simulink library "Lib_Piccolo"  (R2018b)
settings: Solver=VariableStepAuto  StartTime=0.0  StopTime=10.0  RelTol=1e-3
values from neighbouring files (symbols this model uses):
  AccelErrInt2Brakes = 0.15    [SimulationControlConfig16P.m]    (also in SimulationControlConfig16P_LEGACY.m; SimulationControlConfigTAILLESS.m = 0.2; SimulationControlConfigUTAIL.m = 0.2)
  AileronMax = 25    [SimulationControlConfig16P.m]    (also in SimulationControlConfig16P_LEGACY.m; SimulationControlConfigTAILLESS.m; SimulationControlConfigUTAIL.m)
  AileronPower = 0.00268    [SimulationControlConfig16P.m]    (also in SimulationControlConfig16P_LEGACY.m; SimulationControlConfigTAILLESS.m; SimulationControlConfigUTAIL.m)
  AileronSurfaceMax = 45    [SimulationControlConfig16P.m]    (also in SimulationControlConfig16P_LEGACY.m)
  AileronTrim = 0    [SimulationControlConfig16P.m]    (also in SimulationControlConfig16P_LEGACY.m; SimulationControlConfigTAILLESS.m; SimulationControlConfigUTAIL.m)
  Alt = 1000 + TerrainHeight    [SimulationStateConfig.m]
  AltCruise_m = testPlans(testIndx).terrainElevation * 0.3048 + 200    [SimulationControlConfig16P.m]    (also in SimulationControlConfigTAILLESS.m = 1083; SimulationControlConfigUTAIL.m = testPlans(testIndx).terrainElevation * 0.3048 + 152)
  AltitudeRate2PitchCmdIntegratorInit = 0.1    [SimulationControlPre.m]
  AltMax = 10000    [SimulationControlConfig16P.m]    (also in SimulationControlConfig16P_LEGACY.m; SimulationControlConfigTAILLESS.m; SimulationControlConfigUTAIL.m)
  AltMaxAccel = 1.25    [SimulationControlConfig16P.m]    (also in SimulationControlConfig16P_LEGACY.m = 0.9; SimulationControlConfigTAILLESS.m = 1.7; SimulationControlConfigUTAIL.m = 2)
  AltMin = 0    [SimulationControlConfig16P.m]    (also in SimulationControlConfig16P_LEGACY.m; SimulationControlConfigTAILLESS.m; SimulationControlConfigUTAIL.m)
  AltRateCmd2Pitch = 0.50    (= 0.5)    [SimulationControlConfig16P.m]    (also in SimulationControlConfig16P_LEGACY.m = 0.6; SimulationControlConfigTAILLESS.m = 0.2; SimulationControlConfigUTAIL.m = 0.3)
  AltRateError2Pitch = 0.40    (= 0.4)    [SimulationControlConfig16P.m]    (also in SimulationControlConfig16P_LEGACY.m; SimulationControlConfigTAILLESS.m = 0.55; SimulationControlConfigUTAIL.m = 0.55)
  AltRateErrorInt2Pitch = 0.50    (= 0.5)    [SimulationControlConfig16P.m]    (also in SimulationControlConfig16P_LEGACY.m = 0.45; SimulationControlConfigTAILLESS.m; SimulationControlConfigUTAIL.m = 0.75)
  AltRateLpfCutOff = 3    [SimulationControlConfig16P.m]    (also in SimulationControlConfig16P_LEGACY.m; SimulationControlConfigTAILLESS.m = 2; SimulationControlConfigUTAIL.m = 2)
  AutoNosegear2Rudder = 26    [SimulationControlConfig16P.m]    (also in SimulationControlConfig16P_LEGACY.m; SimulationControlConfigTAILLESS.m = 25.2; SimulationControlConfigUTAIL.m = 14)
  b = 5.54    [SimulationControlConfig16P.m]    (also in SimulationControlConfig16P_LEGACY.m; SimulationControlConfigTAILLESS.m = 2.37; SimulationControlConfigUTAIL.m = 2.37)
  Bank2AileronIntegratorInit = 0    [SimulationControlPre.m]
  BankMax_User = BankMax_User/180*pi    (= 0.523598775598)    [SimulationControlConfig16P.m]    (also in SimulationControlConfig16P_LEGACY.m; SimulationControlConfigTAILLESS.m = 0.610865238198; SimulationControlConfigUTAIL.m = 0.628318530718)
  baseLegFlaps = 20    [SimulationControlConfig16P.m]    (also in SimulationControlConfig16P_LEGACY.m = 0; SimulationControlConfigTAILLESS.m = 15; SimulationControlConfigUTAIL.m = 10)
  C = GeneticOpt.C    [SimulationCostFunction.m]
  c = Sw/b    (= 0.841696750903)    [SimulationControlConfig16P.m]    (also in SimulationControlConfig16P_LEGACY.m; SimulationControlConfigTAILLESS.m = 0.354008438819; SimulationControlConfigUTAIL.m = 0.354008438819)
  cell2WheelFactorMG = 5.98    [SimulationSensorConfig16P_LEGACY.m]
  cell2WheelFactorNG = 1    [SimulationSensorConfig16P_LEGACY.m]
  cellSatMaxMG = 15000    [SimulationSensorConfig16P.m]    (also in SimulationSensorConfig16P_LEGACY.m; SimulationSensorConfigTAILLESS7P.m; SimulationSensorConfigUTAIL7P.m)
  cellSatMaxNG = 1000    [SimulationSensorConfig16P.m]    (also in SimulationSensorConfig16P_LEGACY.m; SimulationSensorConfigTAILLESS7P.m; SimulationSensorConfigUTAIL7P.m)
  cellSatMinMG = -15000    [SimulationSensorConfig16P.m]    (also in SimulationSensorConfig16P_LEGACY.m; SimulationSensorConfigTAILLESS7P.m; SimulationSensorConfigUTAIL7P.m)
  cellSatMinNG = -1000    [SimulationSensorConfig16P.m]    (also in SimulationSensorConfig16P_LEGACY.m; SimulationSensorConfigTAILLESS7P.m; SimulationSensorConfigUTAIL7P.m)
  CL_Limit = CL_Max    (= 0.54)    [SimulationControlConfig16P.m]    (also in SimulationControlConfig16P_LEGACY.m; SimulationControlConfigTAILLESS.m; SimulationControlConfigUTAIL.m = 0.53)
  CL_Max = 0.54    [SimulationControlConfig16P.m]    (also in SimulationControlConfig16P_LEGACY.m; SimulationControlConfigTAILLESS.m; SimulationControlConfigUTAIL.m = 0.53)
  CL_Max_Nom = 0.465    [SimulationControlConfig16P.m]    (also in SimulationControlConfig16P_LEGACY.m; SimulationControlConfigTAILLESS.m = 0.39; SimulationControlConfigUTAIL.m)
  CL_Min = 0    [SimulationControlConfig16P.m]    (also in SimulationControlConfig16P_LEGACY.m; SimulationControlConfigTAILLESS.m; SimulationControlConfigUTAIL.m)
  ClimbMaxFraction = 0.35    [SimulationControlConfig16P.m]    (also in SimulationControlConfig16P_LEGACY.m = 0.24; SimulationControlConfigTAILLESS.m = 0.19; SimulationControlConfigUTAIL.m = 0.21)
  ClimboutMaxBank = 7.0    (= 7)    [SimulationControlConfig16P.m]    (also in SimulationControlConfig16P_LEGACY.m; SimulationControlConfigTAILLESS.m = 5; SimulationControlConfigUTAIL.m)
  ClimboutTimer = 7.0    (= 7)    [SimulationControlConfig16P.m]    (also in SimulationControlConfig16P_LEGACY.m; SimulationControlConfigTAILLESS.m; SimulationControlConfigUTAIL.m)
  dCl_per_dFlap = 0.005581818    [SimulationControlConfig16P.m]    (also in SimulationControlConfig16P_LEGACY.m = 0; SimulationControlConfigTAILLESS.m = 0; SimulationControlConfigUTAIL.m = 0)
  DecelerationCmd = 3.1    [SimulationControlConfig16P.m]    (also in SimulationControlConfig16P_LEGACY.m; SimulationControlConfigTAILLESS.m = 0.1; SimulationControlConfigUTAIL.m = 0.1)
  DeRotateLogicEndTimer = abs((NoseDownLimit_Deg-1)/DeRotateRamp_Dps)    [SimulationControlConfig16P.m]    (also in SimulationControlConfig16P_LEGACY.m; SimulationControlConfigTAILLESS.m; SimulationControlConfigUTAIL.m)
  DeRotateLogicHoldNoseUpTimer = 0.1    [SimulationControlConfig16P.m]    (also in SimulationControlConfig16P_LEGACY.m; SimulationControlConfigTAILLESS.m; SimulationControlConfigUTAIL.m)
  DeRotateLogicTimerTimeout = 2    [SimulationControlConfig16P.m]    (also in SimulationControlConfig16P_LEGACY.m; SimulationControlConfigTAILLESS.m; SimulationControlConfigUTAIL.m)
  DeRotateLowerCmdSaturation = 0    [SimulationControlConfig16P.m]    (also in SimulationControlConfig16P_LEGACY.m; SimulationControlConfigTAILLESS.m; SimulationControlConfigUTAIL.m)
  DeRotateRamp_Dps = 3    [SimulationControlConfig16P.m]    (also in SimulationControlConfig16P_LEGACY.m; SimulationControlConfigTAILLESS.m = 8; SimulationControlConfigUTAIL.m = 8)
  DeRotateUpperCmdSaturation = 7    [SimulationControlConfig16P.m]    (also in SimulationControlConfig16P_LEGACY.m; SimulationControlConfigTAILLESS.m; SimulationControlConfigUTAIL.m)
  DescentMaxFraction = 0.22    [SimulationControlConfig16P.m]    (also in SimulationControlConfig16P_LEGACY.m = 0.2; SimulationControlConfigTAILLESS.m = 0.17; SimulationControlConfigUTAIL.m = 0.17)
  DesktopSimTerrainOffset_m = 0.406    [SimulationAircraftConfig.m]
  downwindFlaps = 0    [SimulationControlConfig16P.m]    (also in SimulationControlConfig16P_LEGACY.m; SimulationControlConfigTAILLESS.m; SimulationControlConfigUTAIL.m)
  DP_init = 0.5*1.225*V_init^2    [SimulationControlConfig16P.m]    (also in SimulationControlConfig16P_LEGACY.m; SimulationControlConfigTAILLESS.m; SimulationControlConfigUTAIL.m)
  dscNoiseMG = 1    [SimulationSensorConfig16P_LEGACY.m]
  dscNoiseNG = 0.25    [SimulationSensorConfig16P_LEGACY.m]
  DSCnumBits = 24    [SimulationSensorConfig16P.m]    (also in SimulationSensorConfig16P_LEGACY.m; SimulationSensorConfigTAILLESS7P.m; SimulationSensorConfigUTAIL7P.m)
  DSCRangeMaxMG = 15000    [SimulationSensorConfig16P.m]    (also in SimulationSensorConfig16P_LEGACY.m; SimulationSensorConfigTAILLESS7P.m; SimulationSensorConfigUTAIL7P.m)
  DSCRangeMaxNG = 1000    [SimulationSensorConfig16P.m]    (also in SimulationSensorConfig16P_LEGACY.m; SimulationSensorConfigTAILLESS7P.m; SimulationSensorConfigUTAIL7P.m)
  DSCRangeMinMG = -15000    [SimulationSensorConfig16P.m]    (also in SimulationSensorConfig16P_LEGACY.m; SimulationSensorConfigTAILLESS7P.m; SimulationSensorConfigUTAIL7P.m)
  DSCRangeMinNG = -1000    [SimulationSensorConfig16P.m]    (also in SimulationSensorConfig16P_LEGACY.m; SimulationSensorConfigTAILLESS7P.m; SimulationSensorConfigUTAIL7P.m)
  dt = DLLSim.dt    [SimulationTimeStep.m]    (also in SimulationTrim.m = 0.02)
  EarlyTouchdownThreshold = 3.0    (= 3)    [SimulationControlConfig16P.m]    (also in SimulationControlConfig16P_LEGACY.m; SimulationControlConfigTAILLESS.m = 2.2; SimulationControlConfigUTAIL.m = 2.5)
  ElevatorDeflectionRate = 15    [SimulationControlConfig16P.m]    (also in SimulationControlConfig16P_LEGACY.m = 12; SimulationControlConfigTAILLESS.m = 10; SimulationControlConfigUTAIL.m = 12)
  ElevatorMax = 25    [SimulationControlConfig16P.m]    (also in SimulationControlConfig16P_LEGACY.m; SimulationControlConfigTAILLESS.m; SimulationControlConfigUTAIL.m)
  ElevatorPower = -0.002209    [SimulationControlConfig16P.m]    (also in SimulationControlConfig16P_LEGACY.m; SimulationControlConfigTAILLESS.m = -0.002956; SimulationControlConfigUTAIL.m = -0.00205983)
  ElevatorTrim = -3.5    [SimulationControlConfig16P.m]    (also in SimulationControlConfig16P_LEGACY.m; SimulationControlConfigTAILLESS.m = -6; SimulationControlConfigUTAIL.m = -8)
  elevonBias = 0    [SimulationControlConfig16P.m]    (also in SimulationControlConfig16P_LEGACY.m; SimulationControlConfigTAILLESS.m; SimulationControlConfigUTAIL.m)
  Enable_TAS_Protection = 0    [SimulationControlConfig16P.m]    (also in SimulationControlConfig16P_LEGACY.m; SimulationControlConfigTAILLESS.m; SimulationControlConfigUTAIL.m)
  EnableCrossTrackAbort = 1    [SimulationControlConfig16P.m]    (also in SimulationControlConfigTAILLESS.m; SimulationControlConfigUTAIL.m)
  EnergyBandwidth = 0.02    [SimulationControlConfig16P.m]    (also in SimulationControlConfig16P_LEGACY.m; SimulationControlConfigTAILLESS.m = 0.06; SimulationControlConfigUTAIL.m = 0.06)
  EngineLhFuelCut = 0    [SimulationAircraftConfig.m]
  EngineRhFuelCut = 0    [SimulationAircraftConfig.m]
  FastThrottleRate = 0.075    [SimulationControlConfig16P.m]    (also in SimulationControlConfig16P_LEGACY.m = 0.05; SimulationControlConfigTAILLESS.m = 0.1; SimulationControlConfigUTAIL.m = 0.1)
  FilterWarmUpTime = 2    [SimulationSensorConfig16P.m]    (also in SimulationSensorConfig16P_LEGACY.m; SimulationSensorConfigTAILLESS7P.m; SimulationSensorConfigUTAIL7P.m)
  finalApproachFlaps = 20    [SimulationControlConfig16P.m]    (also in SimulationControlConfig16P_LEGACY.m = 0; SimulationControlConfigTAILLESS.m = 22; SimulationControlConfigUTAIL.m = 10)
  FinalDescentSlope_Deg = testPlans(testIndx).descentSlope    [SimulationControlConfig16P.m]    (also in SimulationControlConfig16P_LEGACY.m; SimulationControlConfigTAILLESS.m; SimulationControlConfigUTAIL.m)
  flapMax = 0    [SimulationControlConfig16P.m]    (also in SimulationControlConfig16P_LEGACY.m; SimulationControlConfigTAILLESS.m; SimulationControlConfigUTAIL.m)
  flapRate = 7.5    [SimulationControlConfig16P.m]    (also in SimulationControlConfig16P_LEGACY.m; SimulationControlConfigTAILLESS.m = 6.6; SimulationControlConfigUTAIL.m)
  FlareHeight = 5    [SimulationControlConfig16P.m]    (also in SimulationControlConfig16P_LEGACY.m = 4.8; SimulationControlConfigTAILLESS.m = 2.5; SimulationControlConfigUTAIL.m = 2)
  FlareVerticalRate_mps = -0.4    [SimulationControlConfig16P.m]    (also in SimulationControlConfig16P_LEGACY.m = -0.5; SimulationControlConfigTAILLESS.m = -0.15; SimulationControlConfigUTAIL.m = -0.15)
  Fp_Aileron = 0.55*2*pi*RollRateLpfCutoff*dt    [SimulationControlConfig16P.m]    (also in SimulationControlConfig16P_LEGACY.m; SimulationControlConfigTAILLESS.m; SimulationControlConfigUTAIL.m)
  Fp_Alt = 0.55*AltBandwidth    (= 0.099)    [SimulationControlConfig16P.m]    (also in SimulationControlConfig16P_LEGACY.m; SimulationControlConfigTAILLESS.m = 0.587477826221; SimulationControlConfigUTAIL.m = 0.69115038379)
  Fp_AltRate = 0.55*2*pi*AltRateLpfCutOff*dt    [SimulationControlConfig16P.m]    (also in SimulationControlConfig16P_LEGACY.m; SimulationControlConfigTAILLESS.m; SimulationControlConfigUTAIL.m)
  Fp_Elevator = 0.55*2*pi*PitchRateLpfCutoff*dt    [SimulationControlConfig16P.m]    (also in SimulationControlConfig16P_LEGACY.m; SimulationControlConfigTAILLESS.m; SimulationControlConfigUTAIL.m)
  Fp_Energy = 0.55*2*pi*EnergyBandwidth    (= 0.069115038379)    [SimulationControlConfig16P.m]    (also in SimulationControlConfig16P_LEGACY.m; SimulationControlConfigTAILLESS.m = 0.207345115137; SimulationControlConfigUTAIL.m = 0.207345115137)
  Fp_Energy2 = 0.55*2*pi*EnergyBandwidth*dt    [SimulationControlConfig16P.m]    (also in SimulationControlConfig16P_LEGACY.m; SimulationControlConfigTAILLESS.m; SimulationControlConfigUTAIL.m)
  Fp_Pitch = 0.55*2*pi*PitchBandwidth    (= 2.76460153516)    [SimulationControlConfig16P.m]    (also in SimulationControlConfig16P_LEGACY.m = 3.11017672705; SimulationControlConfigTAILLESS.m = 3.80132711084; SimulationControlConfigUTAIL.m = 2.41902634326)
  Fp_Pitch_2 = 0.55*2*pi*PitchBandwidth*dt    [SimulationControlConfig16P.m]    (also in SimulationControlConfig16P_LEGACY.m; SimulationControlConfigTAILLESS.m; SimulationControlConfigUTAIL.m)
  Fp_Roll = RollBandwidth^2    (= 1)    [SimulationControlConfig16P.m]    (also in SimulationControlConfig16P_LEGACY.m = 1.44; SimulationControlConfigTAILLESS.m; SimulationControlConfigUTAIL.m)
  Fp_Rudder = 0.55*2*pi*YawRateLpfCutoff*dt    [SimulationControlConfig16P.m]    (also in SimulationControlConfig16P_LEGACY.m; SimulationControlConfigTAILLESS.m; SimulationControlConfigUTAIL.m)
  Fp_TAS = 0.55*2*pi*TASBandwidth    (= 0.103672557568)    [SimulationControlConfig16P.m]    (also in SimulationControlConfig16P_LEGACY.m; SimulationControlConfigTAILLESS.m = 0.172787595947; SimulationControlConfigUTAIL.m = 0.172787595947)
  Fp_TAS_Filter = 2*pi*TasLpfCutoff*dt    [SimulationControlConfig16P.m]    (also in SimulationControlConfig16P_LEGACY.m; SimulationControlConfigTAILLESS.m; SimulationControlConfigUTAIL.m)
  Fp_Turn = 0.55*2*pi*TurnErrLPFcutoff    (= 0.0345575191895)    [SimulationControlConfig16P.m]    (also in SimulationControlConfig16P_LEGACY.m; SimulationControlConfigTAILLESS.m = 0.172787595947; SimulationControlConfigUTAIL.m = 0.172787595947)
  Fp_TurnDerr = 0.55*2*pi*TurnDerivativeLPFcutoff    (= 0.0345575191895)    [SimulationControlConfig16P.m]    (also in SimulationControlConfig16P_LEGACY.m; SimulationControlConfigTAILLESS.m = 0.172787595947; SimulationControlConfigUTAIL.m = 0.172787595947)
  FTV = 3    [SimulationAircraftConfig.m]
  ftvStaticPositionError = 1/1.18    (= 0.847457627119)    [SimulationSensorConfig16P.m]    (also in SimulationSensorConfig16P_LEGACY.m; SimulationSensorConfigTAILLESS7P.m = 1; SimulationSensorConfigUTAIL7P.m = 1)
  g = 9.81    [SimulationStateConfig.m]
  GustSpd_Kts = testPlans(testIndx).gustSpd    [SimulationStateConfig.m]
  GustTriggerVal = testPlans(testIndx).gustTriggerVal    [SimulationStateConfig.m]
  HeadingErr2TurnRate = 0.5    [SimulationControlConfig16P.m]    (also in SimulationControlConfig16P_LEGACY.m; SimulationControlConfigTAILLESS.m; SimulationControlConfigUTAIL.m)
  HeadingErrDer2TurnRate = 0.3    [SimulationControlConfig16P.m]    (also in SimulationControlConfig16P_LEGACY.m; SimulationControlConfigTAILLESS.m; SimulationControlConfigUTAIL.m)
  IASbounce = IASstall*0.8    [SimulationControlPre.m]
  IAScruiseCMD = sqrt(2*m*9.81/(1.225*Sw*CL_cruise))    [SimulationControlConfig16P.m]    (also in SimulationControlConfig16P_LEGACY.m; SimulationControlConfigTAILLESS.m; SimulationControlConfigUTAIL.m)
  IASfinalCMD = 1.12 * IASmin    [SimulationControlConfig16P.m]    (also in SimulationControlConfig16P_LEGACY.m = 1.10 * IASmin; SimulationControlConfigTAILLESS.m = 1.10 * IASmin; SimulationControlConfigUTAIL.m = 1.15 * IASmin)
  IASflareCMD = IASstall    [SimulationControlConfig16P.m]    (also in SimulationControlConfig16P_LEGACY.m; SimulationControlConfigTAILLESS.m; SimulationControlConfigUTAIL.m)
  IASmax = 64    [SimulationControlConfig16P.m]    (also in SimulationControlConfig16P_LEGACY.m = 46; SimulationControlConfigTAILLESS.m = 38.58; SimulationControlConfigUTAIL.m = 35)
  IASmin = sqrt(2*m*9.81/(1.225*Sw*0.9*CL_Max_Nom))    [SimulationControlConfig16P.m]    (also in SimulationControlConfig16P_LEGACY.m; SimulationControlConfigTAILLESS.m; SimulationControlConfigUTAIL.m)
  IASshortCMD = IASstall    [SimulationControlConfig16P.m]    (also in SimulationControlConfig16P_LEGACY.m; SimulationControlConfigTAILLESS.m; SimulationControlConfigUTAIL.m)
  IASstall = sqrt(2*m*9.81/(1.225*Sw*CL_Max))    [SimulationControlConfig16P.m]    (also in SimulationControlConfig16P_LEGACY.m; SimulationControlConfigTAILLESS.m; SimulationControlConfigUTAIL.m)
  inFlight = 1    [SimulationControlConfig16P.m]    (also in SimulationControlConfigTAILLESS.m; SimulationControlConfigUTAIL.m)
  JetCatOffset = 5    [SimulationControlConfig16P.m]    (also in SimulationControlConfig16P_LEGACY.m)
  LaunchRollingElevator = -1.5    [SimulationControlConfig16P.m]    (also in SimulationControlConfig16P_LEGACY.m; SimulationControlConfigTAILLESS.m = 1; SimulationControlConfigUTAIL.m = 1)
  ldg_NosegearMax = 10    [SimulationControlConfig16P.m]    (also in SimulationControlConfig16P_LEGACY.m; SimulationControlConfigTAILLESS.m; SimulationControlConfigUTAIL.m)
  ldg_TrackVyErrInt2Nosegear = 0.1250    (= 0.125)    [SimulationControlConfig16P.m]    (also in SimulationControlConfig16P_LEGACY.m; SimulationControlConfigTAILLESS.m = 0.00714285714286; SimulationControlConfigUTAIL.m = 0.00714285714286)
  ldg_TrackVyErrPro2Nosegear = 0.35    [SimulationControlConfig16P.m]    (also in SimulationControlConfig16P_LEGACY.m; SimulationControlConfigTAILLESS.m = 0.0546666666667; SimulationControlConfigUTAIL.m = 0.0546666666667)
  ldg_TrackY2Vy = 0.07    [SimulationControlConfig16P.m]    (also in SimulationControlConfig16P_LEGACY.m; SimulationControlConfigTAILLESS.m = 0.17; SimulationControlConfigUTAIL.m = 0.17)
  ldg_Vy2NosegearScalingPower = 1.075    [SimulationControlConfig16P.m]    (also in SimulationControlConfig16P_LEGACY.m; SimulationControlConfigTAILLESS.m = 0.6; SimulationControlConfigUTAIL.m = 0.5)
  ldg_Y2VyScalingPower = 0.175    [SimulationControlConfig16P.m]    (also in SimulationControlConfig16P_LEGACY.m; SimulationControlConfigTAILLESS.m = 0; SimulationControlConfigUTAIL.m = 0)
  ldg_YawRate2Nosegear = 0.175    [SimulationControlConfig16P.m]    (also in SimulationControlConfig16P_LEGACY.m; SimulationControlConfigTAILLESS.m = 0.065; SimulationControlConfigUTAIL.m = 0.065)
  LiftSlope = 0.064285    [SimulationControlConfig16P.m]    (also in SimulationControlConfig16P_LEGACY.m; SimulationControlConfigTAILLESS.m = 0.058631; SimulationControlConfigUTAIL.m)
  LPFaileronInit = 0    [SimulationControlPre.m]
  LPFclestInit = 0    [SimulationControlPre.m]
  LPFenergyFFInit = 0    [SimulationControlPre.m]
  LPFtasInit = V_init + 2    [SimulationControlPre.m]
  LPFthrottleInit = ThrottleTrim    [SimulationControlPre.m]
  LPFturnErrInit = 0    [SimulationControlPre.m]
  ... (+115 more)
undefined symbols (not defined in the file or in its folder): abortFlag, alphaHPF, apmDelay, BRWNOUT, CRAWOR, CRAWUR, DiscIntNeverNeededParam, DLLSim, DLLSimStep, ECOMOR, ECOMUR, Fp_Tas, GustTrigger_HeightAgl_m, IPSTAT, LCINTEG, Ldg_Persist_Time, LOWER_FLAGS, MSG_ENABLE, NoiseStd, OLDVAL, OVERRIDE_ENABLE, OVERRIDE_VALUE, REBOOT, reversionEnable, revIASMax, revIASMin, revPitchMax, revPitchMin, revPitchRateMax, revRollMax, revRollRateMax, SAMPLE, SCALON, SensorModel, sigbuilder_block, Sim_Vx, Sim_Vy, Sim_Vz, Sim_Xpos, Sim_Ypos, Sim_Zpos, SYSOR, SYSUR, TARE, TEMPOR, TEMPUR, testIndx, testPlan, testPlans, Trim_piccoloInCmd, Trim_REFSI_FD_IN_nmodeCgShifterCmd_Ft, Trim_REFSI_FD_IN_nmodeFlapLhIBCmd_Deg, Trim_REFSI_FD_IN_nmodeFlapLhOBCmd_Deg, Trim_REFSI_FD_IN_nmodeFlapRhIBCmd_Deg, Trim_REFSI_FD_IN_nmodeFlapRhOBCmd_Deg, Trim_REFSI_FD_IN_nmodeSlatLhCmd_Deg, Trim_REFSI_FD_IN_nmodeSlatRhCmd_Deg, Trim_REFSI_FD_IN_nmodeSplrLhInbdCmd_Deg, Trim_REFSI_FD_IN_nmodeSplrLhOutbdCmd_Deg ... (+5)
libraries: simulink x866, aerolibconvert2 x60, $bdroot x52, aerolibatmos2 x5, dspswit3 x5, simulink_extras x4, dsparch4 x2, Lib_Piccolo_Alt x2, eeGeneralControl x1, dspindex x1
(part 20 of 44)

== system Lib_Piccolo/Altitude Rate to Pitch Command LEGACY DEROTATE/DeRotate Logic rev 2/Timer 2 ==
  Enable/!Rst : Inport
  Compare To Constant1 : simulink/Logic and Bit Operations/Compare To Constant  relop=>  const=0  OutDataTypeStr=uint8
  Compare To Constant2 : simulink/Logic and Bit Operations/Compare To Constant  relop=>=  const=period  OutDataTypeStr=uint8
  Compare To Constant3 : simulink/Logic and Bit Operations/Compare To Constant  relop===  const=0  OutDataTypeStr=boolean
  Discrete-Time Integrator : DiscreteIntegrator  ExternalReset=level  SampleTime=-1  OutDataTypeStr=double  ICPrevOutput=DiscIntNeverNeededParam  ICPrevScaledInput=DiscIntNeverNeededParam
  Expired : Outport
  wires:
  Compare To Constant1/1 -> Discrete-Time Integrator/1
  Compare To Constant2/1 -> Expired/1
  Discrete-Time Integrator/1 -> Compare To Constant2/1
  Enable/!Rst/1 -> Compare To Constant1/1, Compare To Constant3/1
  Compare To Constant3/1 -> Discrete-Time Integrator/2

== system Lib_Piccolo/Altitude Rate to Pitch Command LEGACY DEROTATE/DeRotate Logic rev 2/Timer1 ==
  Enable/!Rst : Inport
  Compare To Constant1 : simulink/Logic and Bit Operations/Compare To Constant  relop=>  const=0  OutDataTypeStr=uint8
  Compare To Constant2 : simulink/Logic and Bit Operations/Compare To Constant  relop=>=  const=period  OutDataTypeStr=uint8
  Compare To Constant3 : simulink/Logic and Bit Operations/Compare To Constant  relop===  const=0  OutDataTypeStr=boolean
  Discrete-Time Integrator : DiscreteIntegrator  ExternalReset=level  SampleTime=-1  OutDataTypeStr=double  ICPrevOutput=DiscIntNeverNeededParam  ICPrevScaledInput=DiscIntNeverNeededParam
  Expired : Outport
  wires:
  Compare To Constant1/1 -> Discrete-Time Integrator/1
  Compare To Constant2/1 -> Expired/1
  Discrete-Time Integrator/1 -> Compare To Constant2/1
  Enable/!Rst/1 -> Compare To Constant1/1, Compare To Constant3/1
  Compare To Constant3/1 -> Discrete-Time Integrator/2

== system Lib_Piccolo/Bank to Aileron/Bank Angle Limit Calculation/User and State Machine Limits  ==
  apMode : Inport
  Compare To Constant1 : simulink/Logic and Bit Operations/Compare To Constant  relop=<=  const=1  OutDataTypeStr=uint8
  Compare To Constant2 : simulink/Logic and Bit Operations/Compare To Constant  relop===  const=3  OutDataTypeStr=uint8
  Compare To Constant3 : simulink/Logic and Bit Operations/Compare To Constant  relop===  const=2  OutDataTypeStr=uint8
  Compare To Constant4 : simulink/Logic and Bit Operations/Compare To Constant  relop===  const=11  OutDataTypeStr=uint8
  Compare To Constant5 : simulink/Logic and Bit Operations/Compare To Constant  relop=>=  const=9  OutDataTypeStr=uint8
  Constant1 : Constant  Value=BankMax_User
  Constant2 : Constant  Value=ClimboutMaxBank*pi/180
  Constant8 : Constant  Value=MaxTouchdownBank*pi/180
  GroundBankCmd : Constant  Value=0
  OR : Logic  Operator=OR  IconShape=distinctive  AllPortsSameDT=off  OutDataTypeStr=boolean
  OR1 : Logic  Operator=OR  IconShape=distinctive  AllPortsSameDT=off  OutDataTypeStr=boolean
  Switch : Switch  Criteria=u2 > Threshold
  Switch3 : Switch  Criteria=u2 > Threshold
  Switch4 : Switch  Criteria=u2 > Threshold
  UserLimit : Outport
  wires:
  Constant2/1 -> Switch4/1
  OR1/1 -> Switch4/2
  Compare To Constant3/1 -> OR1/1
  Compare To Constant2/1 -> OR1/2
  Switch/1 -> UserLimit/1
  Switch3/1 -> Switch4/3
  Switch4/1 -> Switch/3
  Constant8/1 -> Switch3/1
  Constant1/1 -> Switch3/3
  Compare To Constant4/1 -> OR/1
  OR/1 -> Switch/2
  apMode/1 -> Compare To Constant5/1, Compare To Constant4/1, Compare To Constant1/1, Compare To Constant2/1, Compare To Constant3/1
  GroundBankCmd/1 -> Switch/1
  Compare To Constant5/1 -> Switch3/2
  Compare To Constant1/1 -> OR/2

== system Lib_Piccolo/Bank to Aileron/Dynamic Inversion PID/Dimensional Aileron Power ==
  Dynamic Pressure (Avoid Small Value) : Inport
  Multiply : Product  Inputs=****/
  Roll Axis Inertia : Constant  Value=XInertia
  Unit: Per Deg : Constant  Value=AileronPower
  Wing Area : Constant  Value=Sw
  Wing Span : Constant  Value=b
  CP : Outport
  wires:
  Unit: Per Deg/1 -> Multiply/4
  Multiply/1 -> CP/1
  Roll Axis Inertia/1 -> Multiply/5
  Wing Span/1 -> Multiply/3
  Wing Area/1 -> Multiply/2
  Dynamic Pressure (Avoid Small Value)/1 -> Multiply/1

== system Lib_Piccolo/Bank to Aileron/Dynamic Inversion PID/LPF AileronCmd ==
  "Input " : Inport
  Reset : Inport  Port=2
  Add1 : Sum  Inputs=++|
  Compare To Constant2 : simulink/Logic and Bit Operations/Compare To Constant  relop=>  const=0  OutDataTypeStr=uint8
  Constant11 : Constant  Value=RollRateLpfCutoff
  "LPF " : DiscreteTransferFcn  Commented=on  Numerator=[Fp_Aileron 0]  Denominator=[1 Fp_Aileron-1]  InitialStates=LPFaileronInit
  Switch1 : Switch  Criteria=u2 > Threshold
  Unit Delay1 : UnitDelay  InitialCondition=LPFaileronInit  SampleTime=-1
  a1 : Gain  Gain=1-Fp_Aileron
  b0 : Gain  Gain=Fp_Aileron
  Output : Outport
  wires:
  "Input "/1 -> Switch1/3, b0/1
  a1/1 -> Add1/1
  Add1/1 -> Unit Delay1/1, Switch1/1
  b0/1 -> Add1/2
  Unit Delay1/1 -> a1/1
  Switch1/1 -> Output/1
  Compare To Constant2/1 -> Switch1/2
  Constant11/1 -> Compare To Constant2/1

== system Lib_Piccolo/Bank to Aileron/Dynamic Inversion PID/Roll Moment Caused By Damping ==
  note: FWG3 Notes indicated that the RollRate term was absolute and sign should be removed. This is not consistent when matched against Piccolo HW
  RollRate_Body : Inport
  V : Inport  Port=2
  Abs : Abs  Commented=on
  Constant : Constant  Value=RollDamping
  Gain : Gain  Gain=2
  Multiply : Product  Inputs=***/
  Wing Span : Constant  Value=b
  DAMP : Outport
  wires:
  RollRate_Body/1 -> Multiply/2
  Constant/1 -> Multiply/1
  Multiply/1 -> DAMP/1
  Gain/1 -> Multiply/4
  Wing Span/1 -> Multiply/3
  V/1 -> Gain/1

== system Lib_Piccolo/Bank to Aileron/Dynamic Inversion PID/Rollout Roll Control ==
  apMode : Inport
  Aileron In : Inport  Port=2
  AND : Logic  IconShape=distinctive  AllPortsSameDT=off  OutDataTypeStr=boolean
  Compare To Constant1 : simulink/Logic and Bit Operations/Compare To Constant  relop===  const=0  OutDataTypeStr=uint8
  Compare To Constant2 : simulink/Logic and Bit Operations/Compare To Constant  relop=<=  const=0  OutDataTypeStr=uint8
  Compare To Constant3 : simulink/Logic and Bit Operations/Compare To Constant  relop===  const=11  OutDataTypeStr=uint8
  Constant1 : Constant  Value=RolloutWingLeveling
  Constant3 : Constant  Value=0
  OR : Logic  Operator=OR  IconShape=distinctive  AllPortsSameDT=off  OutDataTypeStr=boolean
  Switch1 : Switch  Criteria=u2 > Threshold
  Aileron Out : Outport
  wires:
  Compare To Constant1/1 -> AND/1
  Constant1/1 -> Compare To Constant1/1
  Compare To Constant3/1 -> AND/2
  Aileron In/1 -> Switch1/3
  apMode/1 -> Compare To Constant2/1, Compare To Constant3/1
  AND/1 -> OR/1
  Switch1/1 -> Aileron Out/1
  Constant3/1 -> Switch1/1
  OR/1 -> Switch1/2
  Compare To Constant2/1 -> OR/2

== system Lib_Piccolo/Bank to Aileron/DynamicPLimit/Latch ==
  D : Inport
  Enable/!Rst : Inport  Port=2
  AND : Logic  IconShape=distinctive  AllPortsSameDT=off  OutDataTypeStr=boolean
  Constant : Constant
  OR : Logic  Operator=OR  IconShape=distinctive  AllPortsSameDT=off  OutDataTypeStr=boolean
  Switch : Switch  Criteria=u2 > Threshold  Threshold=0.5
  Unit Delay : UnitDelay  SampleTime=-1
  Q_Latched : Outport
  wires:
  Constant/1 -> Switch/1
  Enable/!Rst/1 -> AND/2
  AND/1 -> Switch/2
  OR/1 -> AND/1
  D/1 -> OR/1, Switch/3
  Switch/1 -> Unit Delay/1, Q_Latched/1
  Unit Delay/1 -> OR/2

== system Lib_Piccolo/Bank to Aileron/Reference Model/Roll Rate Max Accel Rate Limit ==
  note: U(k)
  note: Y(k)
  up : Inport
  u : Inport  Port=2
  lo : Inport  Port=3
  Delay Input2 : UnitDelay  Description=Store in Global RAM  DisableCoverage=on  InitialCondition=RateLimitRollRateAccel  SampleTime=-1
  Difference Inputs1 : Sum  Description=Add in CPU  DisableCoverage=on  Inputs=+-  OutDataTypeStr=Inherit: Inherit via back propagation
  Difference Inputs2 : Sum  Description=Add in CPU  OutDataTypeStr=Inherit: Inherit via back propagation
  FixPt Data Type Duplicate : DataTypeDuplicate  DisableCoverage=on  NumInputPorts=7
  Saturation Dynamic2 : simulink/Discontinuities/Saturation Dynamic  OutMin=[]  OutMax=[]  OutDataTypeStr=Inherit: Same as second input  OutDataType=fixdt(1, 16)  OutScaling=2^-10  DoSatur=off
  delta fall limit : Product  DisableCoverage=on  Inputs=**  OutDataTypeStr=Inherit: Inherit via back propagation  SaturateOnIntegerOverflow=on
  delta rise limit : Product  DisableCoverage=on  Inputs=**  OutDataTypeStr=Inherit: Inherit via back propagation  SaturateOnIntegerOverflow=on
  sample time : SampleTimeMath  DisableCoverage=on  TsampMathOp=Ts Only  weightValue=1
  Y : Outport  InitialOutput=0
  wires:
  delta fall limit/1 -> FixPt Data Type Duplicate/3, Saturation Dynamic2/3
  Difference Inputs1/1 -> FixPt Data Type Duplicate/4, Saturation Dynamic2/2  "( U(k) - Y(k-1) )"
  delta rise limit/1 -> FixPt Data Type Duplicate/6, Saturation Dynamic2/1
  lo/1 -> delta fall limit/1
  Saturation Dynamic2/1 -> Difference Inputs2/1, FixPt Data Type Duplicate/7
  u/1 -> Difference Inputs1/1, FixPt Data Type Duplicate/5, sample time/1
  up/1 -> delta rise limit/1
  Delay Input2/1 -> Difference Inputs2/2, Difference Inputs1/2, FixPt Data Type Duplicate/2  "Y(k-1)"
  sample time/1 -> delta fall limit/2, delta rise limit/2
  Difference Inputs2/1 -> Delay Input2/1, FixPt Data Type Duplicate/1, Y/1

== system Lib_Piccolo/Bank to Aileron/TASLimit/Latch ==
  D : Inport
  Enable/!Rst : Inport  Port=2
  AND : Logic  IconShape=distinctive  AllPortsSameDT=off  OutDataTypeStr=boolean
  Constant : Constant
  OR : Logic  Operator=OR  IconShape=distinctive  AllPortsSameDT=off  OutDataTypeStr=boolean
  Switch : Switch  Criteria=u2 > Threshold  Threshold=0.5
  Unit Delay : UnitDelay  SampleTime=-1
  Q_Latched : Outport
  wires:
  Constant/1 -> Switch/1
  Enable/!Rst/1 -> AND/2
  AND/1 -> Switch/2
  OR/1 -> AND/1
  D/1 -> OR/1, Switch/3
  Switch/1 -> Unit Delay/1, Q_Latched/1
  Unit Delay/1 -> OR/2

== system Lib_Piccolo/Brake Controller/Variant Subsystem/16P ==
  Feedback Bus : Inport
  Bus Selector : BusSelector  OutputSignals=xAccel_Body_mps2
  Clock : Clock
  Compare To Constant : simulink/Logic and Bit Operations/Compare To Constant  relop=>  const=0  OutDataTypeStr=boolean
  Compare To Constant1 : simulink/Logic and Bit Operations/Compare To Constant  relop=>  const=2  OutDataTypeStr=boolean
  Constant : Constant  Value=0
  Constant1 : Constant  Value=PrelaunchBrakes
  Constant7 : Constant  Value=DecelerationCmd
  Gain4 : Gain  Gain=AccelErrInt2Brakes
  Gain5 : Gain  Gain=-1
  Integrator2 : Integrator  ExternalReset=rising
  Saturation1 : Saturate  UpperLimit=1  LowerLimit=0
  Sum4 : Sum  Inputs=|+-
  Switch : Switch  Criteria=u2 > Threshold  Threshold=0.5
  Switch1 : Switch  Criteria=u2 > Threshold  Threshold=0.5
  Brake_Pcnt : Outport
  tag scope: TD_Complete=global, startTaxi=global
  wires:
  Sum4/1 -> Integrator2/1  "accelError"
  Integrator2/1 -> Gain4/1  "errorInt"
  Bus Selector/1 -> Gain5/1  "<xAccel_Body_mps2>"
  Gain5/1 -> Sum4/2  "HWIL.Xaccel"
  Saturation1/1 -> Switch/1  "brakeCtrl"
  Feedback Bus/1 -> Bus Selector/1
  Constant7/1 -> Sum4/1  "TargetXaccel"
  Gain4/1 -> Saturation1/1
  Compare To Constant/1 -> Integrator2/2, Switch/2
  Constant/1 -> Switch/3
  [Rollout_Flag] -> Compare To Constant/1
  [TouchdownDetectedFlag] -> [TD_Complete]  "TD_Flag"
  [startTaxi] -> Switch1/2
  Clock/1 -> Compare To Constant1/1
  Constant1/1 -> Switch1/3
  Switch1/1 -> Brake_Pcnt/1
  Switch/1 -> Switch1/1  "Sim.BrakeCmd"
  Compare To Constant1/1 -> [startTaxi]

== system Lib_Piccolo/Brake Controller/Variant Subsystem/7P ==
  Feedback Bus : Inport
  Clock : Clock
  Compare To Constant1 : simulink/Logic and Bit Operations/Compare To Constant  relop=>  const=2  OutDataTypeStr=boolean
  Constant : Constant  Value=0
  Terminator : Terminator
  Brake_Pcnt : Outport
  tag scope: startTaxi=global
  wires:
  Constant/1 -> Brake_Pcnt/1
  Feedback Bus/1 -> Terminator/1
  Clock/1 -> Compare To Constant1/1
  Compare To Constant1/1 -> [startTaxi]

== system Lib_Piccolo/Control Allocation/M2 Flap-to-Drag /Variant Model ==
  note: 1) Add Subsystem or Model blocks as valid variant choices.
      | 2) You cannot connect blocks at this level. At simulation, connectivity is automatically
      | determined, based on the active variant and port name matching.
  Sim_ThrottleCmd : Inport
  16P5 : Subsystem  VariantControl="modelScale == \"16P5\""
  7P : Subsystem  VariantControl="modelScale == \"7P\""
  ThrottleCmdOut : Outport

== system Lib_Piccolo/Control Allocation/M2_OLD/Variant Model ==
  note: 1) Add Subsystem or Model blocks as valid variant choices.
      | 2) You cannot connect blocks at this level. At simulation, connectivity is automatically
      | determined, based on the active variant and port name matching.
  Sim_ThrottleCmd : Inport
  16P5 : Subsystem  VariantControl="modelScale == \"16P5\""
  7P : Subsystem  VariantControl="modelScale == \"7P\""
  ThrottleCmdOut : Outport

== system Lib_Piccolo/Control Allocation/M7/Variant Model ==
  note: 1) Add Subsystem or Model blocks as valid variant choices.
      | 2) You cannot connect blocks at this level. At simulation, connectivity is automatically
      | determined, based on the active variant and port name matching.
  Sim_ThrottleCmd : Inport
  16P5 : Subsystem  VariantControl="modelScale == \"16P5\""
  7P : Subsystem  VariantControl="modelScale == \"7P\""
  ThrottleCmdOut : Outport

== system Lib_Piccolo/Control Allocation/M8/Variant Model ==
  note: 1) Add Subsystem or Model blocks as valid variant choices.
      | 2) You cannot connect blocks at this level. At simulation, connectivity is automatically
      | determined, based on the active variant and port name matching.
  Sim_ThrottleCmd : Inport
  16P5 : Subsystem  VariantControl="modelScale == \"16P5\""
  7P : Subsystem  VariantControl="modelScale == \"7P\""
  ThrottleCmdOut : Outport

== system Lib_Piccolo/Control Allocation/M8 Flap-to-Drag/Variant Model ==
  note: 1) Add Subsystem or Model blocks as valid variant choices.
      | 2) You cannot connect blocks at this level. At simulation, connectivity is automatically
      | determined, based on the active variant and port name matching.
  Sim_ThrottleCmd : Inport
  16P5 : Subsystem  VariantControl="modelScale == \"16P5\""
  7P : Subsystem  VariantControl="modelScale == \"7P\""
  ThrottleCmdOut : Outport

== system Lib_Piccolo/Control Allocation LEGACY/Variant Model/16P5 ==
  note: Piccolo Thrust Mapping to JetCat at Idle.
  Sim_ThrottleCmd : Inport
  Constant : Constant  Value=100/(100-3)*3
  Decimal to Pct : Gain  Gain=100
  Decimal to Pct1 : Gain  Gain=1/100
  Gain8 : Gain  Gain=100/(100-3)
  Saturation : Saturate  UpperLimit=100  LowerLimit=0
  Sum1 : Sum  Inputs=|+-
  Terminator : Terminator
  ThrottleCmdOut : Outport
  wires:
  Saturation/1 -> ThrottleCmdOut/1, Decimal to Pct1/1
  Gain8/1 -> Sum1/1
  Decimal to Pct1/1 -> Terminator/1  "JetCatCmd"
  Constant/1 -> Sum1/2
  Sim_ThrottleCmd/1 -> Decimal to Pct/1
  Decimal to Pct/1 -> Gain8/1
  Sum1/1 -> Saturation/1

== system Lib_Piccolo/Control Allocation LEGACY/Variant Model/7P ==
  note: Piccolo Thrust Mapping to Ducted Fans
  Sim_ThrottleCmd : Inport
  Decimal to Pct1 : Gain  Gain=1/100
  Saturation : Saturate  UpperLimit=1  LowerLimit=0
  Terminator : Terminator
  ThrottleCmdOut : Outport
  wires:
  Sim_ThrottleCmd/1 -> Saturation/1
  Decimal to Pct1/1 -> Terminator/1  "JetCatCmd"
  Saturation/1 -> ThrottleCmdOut/1, Decimal to Pct1/1

== system Lib_Piccolo/DSC Load Conversion/DSC-to-Wheel MGL/DSC-to-Wheel Global Linear Scaling ==
  DSC_Load_N : Inport
  Constant : Constant  Value=SensorModel.WOW.Cell.gblOffset  OutDataTypeStr=single
  Gain : Gain  Gain=SensorModel.WOW.Cell.gblSlope  OutDataTypeStr=single
  Sum : Sum  Inputs=|++
  WOW_N : Outport  OutDataTypeStr=single  VectorParamsAs1DForOutWhenUnconnected=on
  wires:
  DSC_Load_N/1 -> Gain/1
  Gain/1 -> Sum/1
  Sum/1 -> WOW_N/1
  Constant/1 -> Sum/2

== system Lib_Piccolo/DSC Load Conversion/DSC-to-Wheel MGL/DSC-to-Wheel Polynomial Scaling MGL ==
  DSC_Load_N : Inport  OutDataTypeStr=single
  Square : Math  Operator=square  SaturateOnIntegerOverflow=on
  Sum : Sum  Inputs=+++
  a : Gain  Gain=SensorModel.WOW.Cell.polyA.MGL  OutDataTypeStr=single
  b : Gain  Gain=SensorModel.WOW.Cell.polyB.MGL  OutDataTypeStr=single
  c : Constant  Value=SensorModel.WOW.Cell.polyC.MGL  OutDataTypeStr=single
  WOW_N : Outport  OutDataTypeStr=single  VectorParamsAs1DForOutWhenUnconnected=on
  wires:
  DSC_Load_N/1 -> Square/1, b/1
  a/1 -> Sum/1
  b/1 -> Sum/2
  Square/1 -> a/1
  c/1 -> Sum/3
  Sum/1 -> WOW_N/1

== system Lib_Piccolo/DSC Load Conversion/DSC-to-Wheel MGR/DSC-to-Wheel Global Linear Scaling ==
  DSC_Load_N : Inport
  Constant : Constant  Value=SensorModel.WOW.Cell.gblOffset  OutDataTypeStr=single
  Gain : Gain  Gain=SensorModel.WOW.Cell.gblSlope  OutDataTypeStr=single
  Sum : Sum  Inputs=|++
  WOW_N : Outport  OutDataTypeStr=single  VectorParamsAs1DForOutWhenUnconnected=on
  wires:
  DSC_Load_N/1 -> Gain/1
  Gain/1 -> Sum/1
  Sum/1 -> WOW_N/1
  Constant/1 -> Sum/2

== system Lib_Piccolo/DSC Load Conversion/DSC-to-Wheel MGR/DSC-to-Wheel Polynomial Scaling MGR ==
  DSC_Load_N : Inport  OutDataTypeStr=single
  Square : Math  Operator=square  SaturateOnIntegerOverflow=on
  Sum : Sum  Inputs=+++
  a : Gain  Gain=SensorModel.WOW.Cell.polyA.MGR  OutDataTypeStr=single
  b : Gain  Gain=SensorModel.WOW.Cell.polyB.MGR  OutDataTypeStr=single
  c : Constant  Value=SensorModel.WOW.Cell.polyC.MGR  OutDataTypeStr=single
  WOW_N : Outport  OutDataTypeStr=single  VectorParamsAs1DForOutWhenUnconnected=on
  wires:
  DSC_Load_N/1 -> Square/1, b/1
  a/1 -> Sum/1
  b/1 -> Sum/2
  Square/1 -> a/1
  c/1 -> Sum/3
  Sum/1 -> WOW_N/1

== system Lib_Piccolo/DSC Load Conversion/DSC-to-Wheel NG/DSC-to-Wheel Polynomial Scaling NG ==
  DSC_Load_N : Inport  OutDataTypeStr=single
  Square : Math  Operator=square  SaturateOnIntegerOverflow=on
  Sum : Sum  Inputs=+++
  a : Gain  Gain=SensorModel.WOW.Cell.polyA.NG  OutDataTypeStr=single
  b : Gain  Gain=SensorModel.WOW.Cell.polyB.NG  OutDataTypeStr=single
  c : Constant  Value=SensorModel.WOW.Cell.polyC.NG  OutDataTypeStr=single
  WOW_N : Outport  OutDataTypeStr=single  VectorParamsAs1DForOutWhenUnconnected=on
  wires:
  DSC_Load_N/1 -> Square/1, b/1
  a/1 -> Sum/1
  b/1 -> Sum/2
  Square/1 -> a/1
  c/1 -> Sum/3
  Sum/1 -> WOW_N/1

== system Lib_Piccolo/Emulated INS/Accelerometer Noise Model/Generate Accel Noise ==
  ContactBool : Inport
  gndSpeed_mps : Inport  Port=2
  Constant1 : Constant
  Constant2 : Constant  Value=10
  Data Type Conversion : DataTypeConversion
  Divide : Product  Inputs=*/
  Low-Pass Filter (Discrete or Continuous) : eeGeneralControl/Low-Pass Filter (Discrete or Continuous)  Commented=through  K=1  T=0.2  B=inf  A=-inf  init_option=Inherited from block input  x0=0  Ts=-1
  Multiply{,1..8} (9 alike) : Product
  Saturation3 : Saturate  UpperLimit=SensorModel.IMU.noiseScalarMax  LowerLimit=SensorModel.IMU.noiseScalarMin
  Sum : Sum  Inputs=+-|
  Sum1 : Sum
  Sum2 : Sum
  Sum3 : Sum
  xAccelNoiseInAir : RandomNumber  Variance=SensorModel.IMU.xAccelNoiseVarianceInAir
  xAccelNoiseOnGnd : RandomNumber  Variance=SensorModel.IMU.xAccelNoiseVarianceOnGnd
  yAccelNoiseInAir : RandomNumber  Variance=SensorModel.IMU.yAccelNoiseVarianceInAir
  yAccelNoiseOnGnd : RandomNumber  Variance=SensorModel.IMU.yAccelNoiseVarianceOnGnd
  zAccelNoiseInAir : RandomNumber  Variance=SensorModel.IMU.zAccelNoiseVarianceInAir
  zAccelNoiseOnGnd : RandomNumber  Variance=SensorModel.IMU.zAccelNoiseVarianceOnGnd
  NoiseXaccelmps2 : Outport
  NoiseYaccelmps2 : Outport  Port=2
  NoiseZaccelmps2 : Outport  Port=3
  wires:
  Sum1/1 -> Multiply8/1
  Multiply8/1 -> NoiseXaccelmps2/1
  Multiply7/1 -> NoiseYaccelmps2/1
  Sum2/1 -> Multiply7/1
  Multiply6/1 -> NoiseZaccelmps2/1
  Sum3/1 -> Multiply6/1
  Saturation3/1 -> Multiply6/2, Multiply7/2, Multiply8/2  "gndSpdScalar"
  Constant2/1 -> Divide/2
  Divide/1 -> Saturation3/1
  gndSpeed_mps/1 -> Divide/1
  ContactBool/1 -> Data Type Conversion/1
  Data Type Conversion/1 -> Low-Pass Filter (Discrete or Continuous)/1
  zAccelNoiseInAir/1 -> Multiply4/1
  Multiply5/1 -> Sum3/2
  Multiply4/1 -> Sum3/1
  zAccelNoiseOnGnd/1 -> Multiply5/2
  Multiply2/1 -> Sum2/1
  yAccelNoiseOnGnd/1 -> Multiply3/2
  yAccelNoiseInAir/1 -> Multiply2/1
  Multiply3/1 -> Sum2/2
  xAccelNoiseOnGnd/1 -> Multiply1/2
  xAccelNoiseInAir/1 -> Multiply/1
  Multiply1/1 -> Sum1/2
  Constant1/1 -> Sum/1
  Low-Pass Filter (Discrete or Continuous)/1 -> Sum/2, Multiply1/1, Multiply3/1, Multiply5/1  "onGnd"
  Sum/1 -> Multiply2/2, Multiply4/2, Multiply/2  "inAir"
  Multiply/1 -> Sum1/1

== system Lib_Piccolo/Ground Detection Systems/CL Detection Wrapper/CL Based Touchdown Detection Logic ==
  note: This is a latch used only in the touchdown, and rollout Piccolo Controller Modes
  note: When this is true Piccolo is indicating the WOW system armed.
  note: This is a latch used only in the short final, touchdown, and rollout Piccolo Controller Modes
  Pic_WOW : Inport
  Pic_APMode : Inport  Port=2
  CL : Inport  Port=3
  Compare To Constant1 : simulink/Logic and Bit Operations/Compare To Constant  relop=>  const=-1  OutDataTypeStr=uint8
  Compare To Constant2 : simulink/Logic and Bit Operations/Compare To Constant  relop=>=  const=10  OutDataTypeStr=uint8
  Compare To Constant6 : simulink/Logic and Bit Operations/Compare To Constant  relop=>=  const=9  OutDataTypeStr=uint8
  Constant : Constant  Value=EarlyTouchdownThreshold
  Constant1 : Constant  Value=TouchdownThreshold
  Constant10 : Constant  Value=0
  Constant2 : Constant  Value=CL_Max
  Constant3 : Constant  Value=0
  Constant4 : Constant
  Constant5 : Constant
  Constant6 : Constant  Value=0
  Constant7 : Constant  Value=TouchdownThreshold
  Constant8 : Constant  Value=2
  Constant9 : Constant
  Latch : Subsystem
  Latch1 : Subsystem
  Multiply{,1..4} (5 alike) : Product
  NOT : Logic  Operator=NOT  IconShape=distinctive  AllPortsSameDT=off  OutDataTypeStr=boolean
  Subtract : Sum  Inputs=-+
  Subtract1 : Sum  Inputs=-+
  Subtract2 : Sum  Inputs=+-
  Switch : Switch
  Switch1 : Switch
  Switch2 : Switch  Threshold=2
  Switch3 : Switch
  Switch4 : Switch  Criteria=u2 > Threshold
  EarlyTouchdownFlag : Outport
  TouchdownFlag : Outport  Port=2
  wires:
  Pic_WOW/1 -> Compare To Constant1/1
  Compare To Constant1/1 -> NOT/1
  Switch/1 -> Switch4/1
  Switch3/1 -> Switch4/3
  Constant5/1 -> Switch1/1
  Constant6/1 -> Switch1/3
  Constant4/1 -> Switch/1
  Multiply/1 -> Subtract1/1
  Constant1/1 -> Multiply1/2
  Constant/1 -> Multiply/2
  Constant3/1 -> Switch/3
  Subtract/1 -> Switch/2
  Subtract1/1 -> Switch1/2
  CL/1 -> Subtract2/1, Subtract1/2, Subtract/2
  Constant2/1 -> Multiply/1, Multiply2/1, Multiply1/1
  Multiply1/1 -> Subtract/1
  Constant7/1 -> Switch2/1, Switch2/2
  Switch2/1 -> Multiply2/2
  Multiply2/1 -> Subtract2/2
  Subtract2/1 -> Switch3/2
  Constant9/1 -> Switch3/1
  Constant10/1 -> Switch3/3
  Pic_APMode/1 -> Compare To Constant2/1, Compare To Constant6/1
  Switch1/1 -> Multiply3/1
  Constant8/1 -> Switch2/3
  NOT/1 -> Switch4/2
  Latch/1(Q_Latched) -> EarlyTouchdownFlag/1
  Latch1/1(Q_Latched) -> TouchdownFlag/1
  Compare To Constant2/1 -> Latch1/2(Enable/!Rst), Multiply4/2
  Compare To Constant6/1 -> Latch/2(Enable/!Rst), Multiply3/2
  Multiply3/1 -> Latch/1(D)
  Multiply4/1 -> Latch1/1(D)
  Switch4/1 -> Multiply4/1
